simulink model "state_feedback"  (R2025b)
settings: Solver=ode45  StartTime=0.0  StopTime=10.0  MaxStep=0.001  RelTol=1e-3
undefined symbols (not defined in the file or in its folder): p
settings Model: Creator=Dawid  LastModifiedBy=Dawid

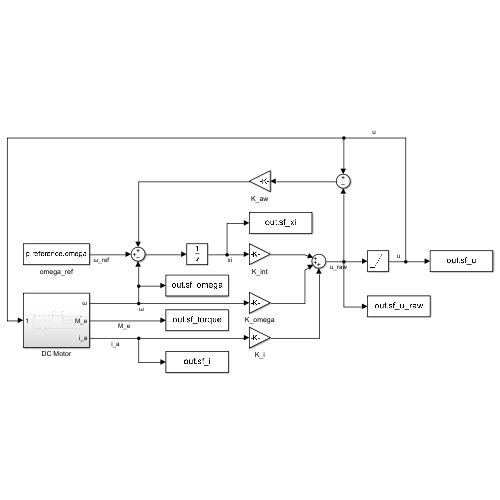
[thumbnail: Simulink's stored preview of the top-level diagram]
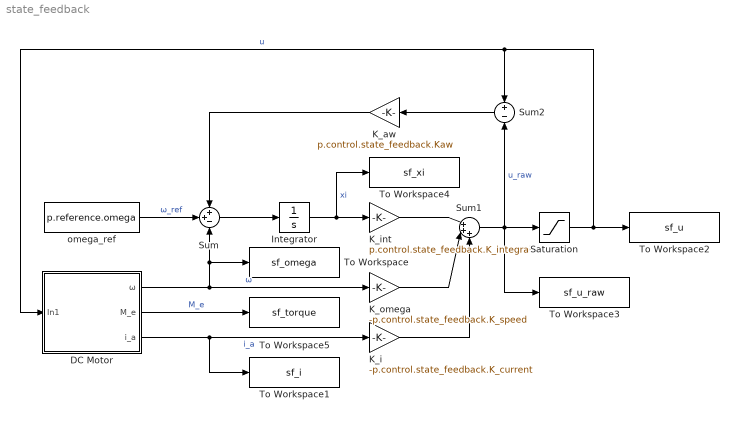
== system state_feedback ==
  DC Motor : Subsystem
  Integrator : Integrator  InitialCondition=p.control.state_feedback.xi0
  K_aw : Gain  Gain=p.control.state_feedback.Kaw
  K_i : Gain  Gain=-p.control.state_feedback.K_current
  K_int : Gain  Gain=p.control.state_feedback.K_integral
  K_omega : Gain  Gain=-p.control.state_feedback.K_speed
  Saturation : Saturate  UpperLimit=p.limits.Umax  LowerLimit=p.limits.Umin
  Sum : Sum  Inputs=++-
  Sum1 : Sum  Inputs=|+++
  Sum2 : Sum  Inputs=+-
  To Workspace : ToWorkspace  VariableName=sf_omega  SaveFormat=Timeseries  SampleTime=-1
  To Workspace1 : ToWorkspace  VariableName=sf_i  SaveFormat=Timeseries  SampleTime=-1
  To Workspace2 : ToWorkspace  VariableName=sf_u  SaveFormat=Timeseries  SampleTime=-1
  To Workspace3 : ToWorkspace  VariableName=sf_u_raw  SaveFormat=Timeseries  SampleTime=-1
  To Workspace4 : ToWorkspace  VariableName=sf_xi  SaveFormat=Timeseries  SampleTime=-1
  To Workspace5 : ToWorkspace  VariableName=sf_torque  SaveFormat=Timeseries  SampleTime=-1
  omega_ref : Constant  Value=p.reference.omega
  wires:
  Sum/1 -> Integrator/1
  Integrator/1 -> To Workspace4/1, K_int/1  "xi"
  DC Motor/3(i_a) -> To Workspace1/1, K_i/1  "i_a"
  DC Motor/1(ω) -> To Workspace/1, Sum/3, K_omega/1  "ω"
  K_int/1 -> Sum1/1
  Sum1/1 -> To Workspace3/1, Sum2/2, Saturation/1  "u_raw"
  Saturation/1 -> To Workspace2/1, Sum2/1, DC Motor/1(In1)  "u"
  K_omega/1 -> Sum1/2
  K_i/1 -> Sum1/3
  DC Motor/2(M_e) -> To Workspace5/1  "M_e"
  Sum2/1 -> K_aw/1
  K_aw/1 -> Sum/1
  omega_ref/1 -> Sum/2  "ω_ref"

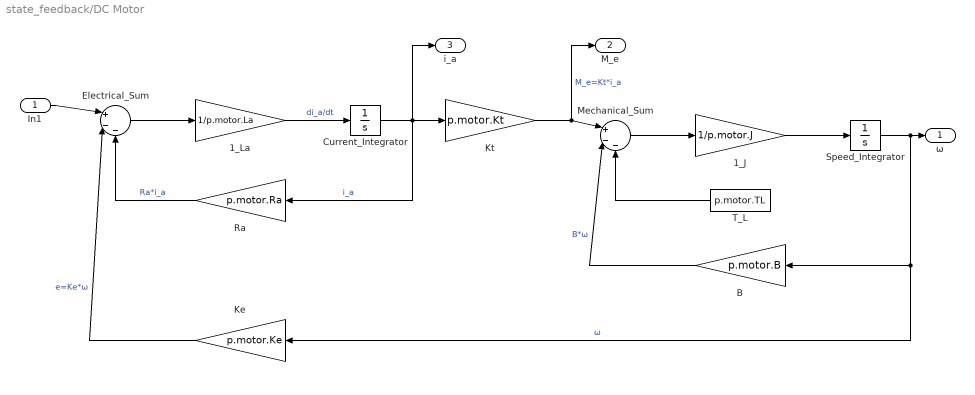
== system state_feedback/DC Motor ==
  In1 : Inport
  1_J : Gain  Gain=1/p.motor.J
  1_La : Gain  Gain=1/p.motor.La
  B : Gain  Gain=p.motor.B
  Current_Integrator : Integrator  InitialCondition=p.initial.i_a
  Electrical_Sum : Sum  Inputs=|+--
  Ke : Gain  Gain=p.motor.Ke
  Kt : Gain  Gain=p.motor.Kt
  Mechanical_Sum : Sum  Inputs=|+--
  Ra : Gain  Gain=p.motor.Ra
  Speed_Integrator : Integrator  InitialCondition=p.initial.omega
  T_L : Constant  Value=p.motor.TL
  ω : Outport
  M_e : Outport  Port=2
  i_a : Outport  Port=3
  wires:
  Speed_Integrator/1 -> B/1, Ke/1, ω/1  "ω"
  Current_Integrator/1 -> i_a/1, Kt/1, Ra/1  "i_a"
  T_L/1 -> Mechanical_Sum/3
  Kt/1 -> M_e/1, Mechanical_Sum/1  "M_e=Kt*i_a"
  1_La/1 -> Current_Integrator/1  "di_a/dt"
  Electrical_Sum/1 -> 1_La/1
  Ra/1 -> Electrical_Sum/3  "Ra*i_a"
  Mechanical_Sum/1 -> 1_J/1
  1_J/1 -> Speed_Integrator/1
  B/1 -> Mechanical_Sum/2  "B*ω"
  Ke/1 -> Electrical_Sum/2  "e=Ke*ω"
  In1/1 -> Electrical_Sum/1
